simulink model "hk_ac_elec_load_rt_2024b"  (R2024b)
settings: Solver=FixedStepAuto  StartTime=0.0  StopTime=inf  FixedStep=1  RelTol=1e-3
libraries: Links_CHRU34207S_Lib x32, simulink x1
settings Model: Creator=Administrator  LastModifiedBy=gao
settings OptimizationCC: BlockReduction=off  ReuseModelBlockBuffer=off
settings HardwareCC: ProdBitPerLong=64  ProdHWDeviceType=Intel->x86-64 (Linux 64)
settings RTWCC: SystemTargetFile=links_rtlnx_grt.tlc  TemplateMakefile=links_rtlnx_grt.tmf  GPUComputeCapability=3.5
settings STFCustomTargetCC: TargetLangStandard=C99 (ISO)  CombineOutputUpdateFcns=on  SystemTargetFile=links_rtlnx_grt.tlc
settings GRTTargetCC: ParMdlRefBuildCompliant=off  CompOptLevelCompliant=off  ConcurrentExecutionCompliant=off  MatFileLogging=off  CPPClassGenCompliant=off  UseToolchainInfoCompliant=off  RTWCAPISignals=on  RTWCAPIParams=on  RTWCAPIRootIO=on
settings ConfigComp: CovMetricSettings=de  CovBoundaryAbsTol=1.0e-5

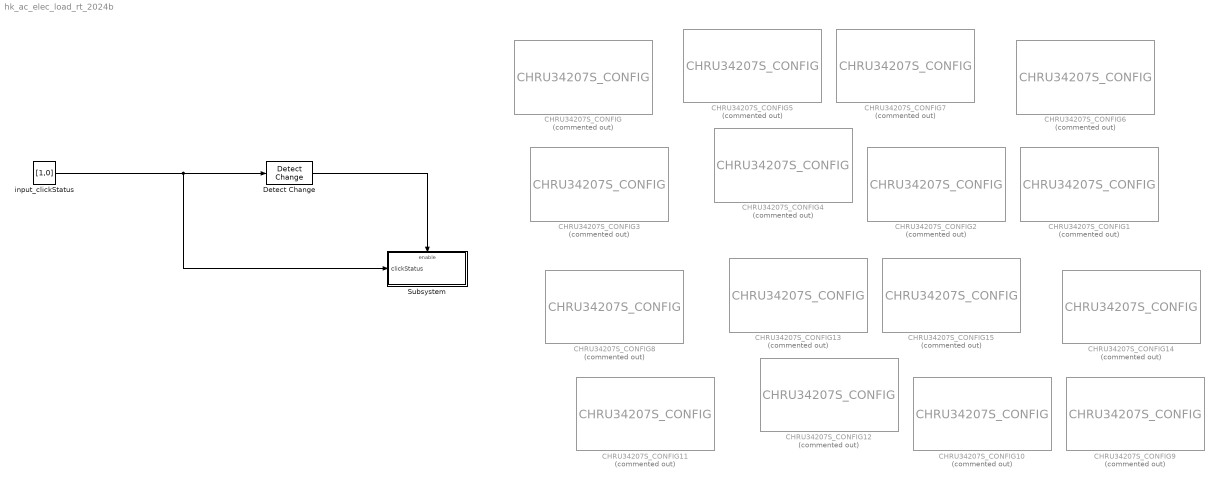
== system hk_ac_elec_load_rt_2024b ==
  CHRU34207S_CONFIG : Links_CHRU34207S_Lib/CHRU34207S_CONFIG  Commented=on  Card=0  Channel=0  Mode=RS422  Baud=115200  Parity=None  DataBits=8  StopBits=1  SampleTime=-1
      settings: SourceProductName=Links_LnxLib
  CHRU34207S_CONFIG1 : Links_CHRU34207S_Lib/CHRU34207S_CONFIG  Commented=on  Card=0  Channel=7  Mode=RS422  Baud=115200  Parity=None  DataBits=8  StopBits=1  SampleTime=-1
      settings: SourceProductName=Links_LnxLib
  CHRU34207S_CONFIG10 : Links_CHRU34207S_Lib/CHRU34207S_CONFIG  Commented=on  Card=0  Channel=14  Mode=RS422  Baud=115200  Parity=None  DataBits=8  StopBits=1  SampleTime=-1
      settings: SourceProductName=Links_LnxLib
  CHRU34207S_CONFIG11 : Links_CHRU34207S_Lib/CHRU34207S_CONFIG  Commented=on  Card=0  Channel=12  Mode=RS422  Baud=115200  Parity=None  DataBits=8  StopBits=1  SampleTime=-1
      settings: SourceProductName=Links_LnxLib
  CHRU34207S_CONFIG12 : Links_CHRU34207S_Lib/CHRU34207S_CONFIG  Commented=on  Card=0  Channel=13  Mode=RS422  Baud=115200  Parity=None  DataBits=8  StopBits=1  SampleTime=-1
      settings: SourceProductName=Links_LnxLib
  CHRU34207S_CONFIG13 : Links_CHRU34207S_Lib/CHRU34207S_CONFIG  Commented=on  Card=0  Channel=9  Mode=RS422  Baud=115200  Parity=None  DataBits=8  StopBits=1  SampleTime=-1
      settings: SourceProductName=Links_LnxLib
  CHRU34207S_CONFIG14 : Links_CHRU34207S_Lib/CHRU34207S_CONFIG  Commented=on  Card=0  Channel=11  Mode=RS422  Baud=115200  Parity=None  DataBits=8  StopBits=1  SampleTime=-1
      settings: SourceProductName=Links_LnxLib
  CHRU34207S_CONFIG15 : Links_CHRU34207S_Lib/CHRU34207S_CONFIG  Commented=on  Card=0  Channel=10  Mode=RS422  Baud=115200  Parity=None  DataBits=8  StopBits=1  SampleTime=-1
      settings: SourceProductName=Links_LnxLib
  CHRU34207S_CONFIG2 : Links_CHRU34207S_Lib/CHRU34207S_CONFIG  Commented=on  Card=0  Channel=6  Mode=RS422  Baud=115200  Parity=None  DataBits=8  StopBits=1  SampleTime=-1
      settings: SourceProductName=Links_LnxLib
  CHRU34207S_CONFIG3 : Links_CHRU34207S_Lib/CHRU34207S_CONFIG  Commented=on  Card=0  Channel=4  Mode=RS422  Baud=115200  Parity=None  DataBits=8  StopBits=1  SampleTime=-1
      settings: SourceProductName=Links_LnxLib
  CHRU34207S_CONFIG4 : Links_CHRU34207S_Lib/CHRU34207S_CONFIG  Commented=on  Card=0  Channel=5  Mode=RS422  Baud=115200  Parity=None  DataBits=8  StopBits=1  SampleTime=-1
      settings: SourceProductName=Links_LnxLib
  CHRU34207S_CONFIG5 : Links_CHRU34207S_Lib/CHRU34207S_CONFIG  Commented=on  Card=0  Channel=1  Mode=RS422  Baud=115200  Parity=None  DataBits=8  StopBits=1  SampleTime=-1
      settings: SourceProductName=Links_LnxLib
  CHRU34207S_CONFIG6 : Links_CHRU34207S_Lib/CHRU34207S_CONFIG  Commented=on  Card=0  Channel=3  Mode=RS422  Baud=115200  Parity=None  DataBits=8  StopBits=1  SampleTime=-1
      settings: SourceProductName=Links_LnxLib
  CHRU34207S_CONFIG7 : Links_CHRU34207S_Lib/CHRU34207S_CONFIG  Commented=on  Card=0  Channel=2  Mode=RS422  Baud=115200  Parity=None  DataBits=8  StopBits=1  SampleTime=-1
      settings: SourceProductName=Links_LnxLib
  CHRU34207S_CONFIG8 : Links_CHRU34207S_Lib/CHRU34207S_CONFIG  Commented=on  Card=0  Channel=8  Mode=RS422  Baud=115200  Parity=None  DataBits=8  StopBits=1  SampleTime=-1
      settings: SourceProductName=Links_LnxLib
  CHRU34207S_CONFIG9 : Links_CHRU34207S_Lib/CHRU34207S_CONFIG  Commented=on  Card=0  Channel=15  Mode=RS422  Baud=115200  Parity=None  DataBits=8  StopBits=1  SampleTime=-1
      settings: SourceProductName=Links_LnxLib
  Detect Change : simulink/Logic and Bit Operations/Detect Change  vinit=[0,0]  OutDataTypeStr=boolean
  Subsystem : Subsystem
  input_clickStatus : Constant  Value=[1,0]  VectorParams1D=off
  wires:
  input_clickStatus/1 -> Subsystem/1(clickStatus), Detect Change/1
  Detect Change/1 -> Subsystem/Enable

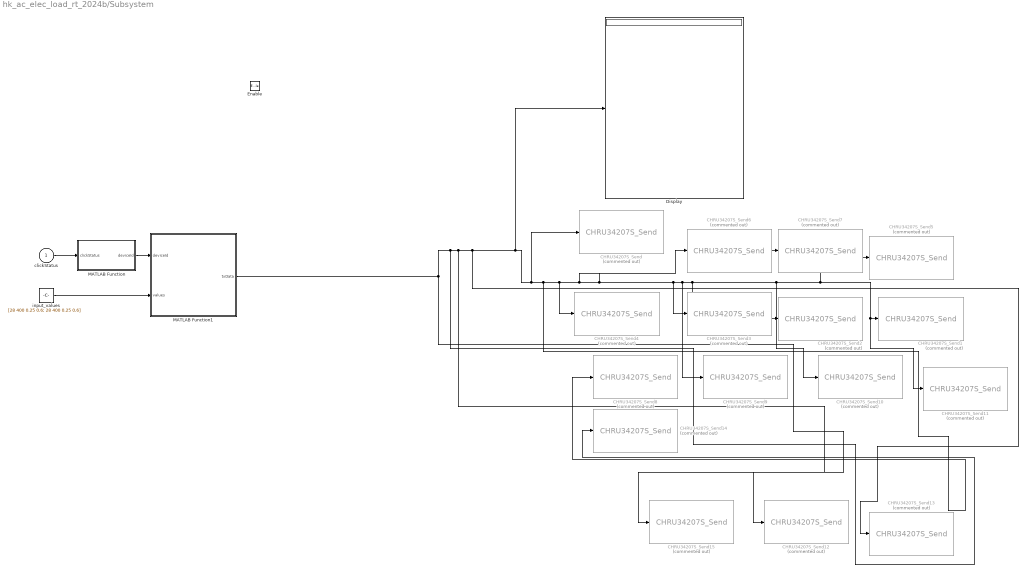
== system hk_ac_elec_load_rt_2024b/Subsystem ==
  clickStatus : Inport
  Enable : EnablePort
  CHRU34207S_Send : Links_CHRU34207S_Lib/CHRU34207S_Send  Commented=on  Card=0  Channel=0  SampleTime=-1
      settings: SourceProductName=Links_LnxLib
  CHRU34207S_Send1 : Links_CHRU34207S_Lib/CHRU34207S_Send  Commented=on  Card=0  Channel=7  SampleTime=-1
      settings: SourceProductName=Links_LnxLib
  CHRU34207S_Send10 : Links_CHRU34207S_Lib/CHRU34207S_Send  Commented=on  Card=0  Channel=10  SampleTime=-1
      settings: SourceProductName=Links_LnxLib
  CHRU34207S_Send11 : Links_CHRU34207S_Lib/CHRU34207S_Send  Commented=on  Card=0  Channel=11  SampleTime=-1
      settings: SourceProductName=Links_LnxLib
  CHRU34207S_Send12 : Links_CHRU34207S_Lib/CHRU34207S_Send  Commented=on  Card=0  Channel=14  SampleTime=-1
      settings: SourceProductName=Links_LnxLib
  CHRU34207S_Send13 : Links_CHRU34207S_Lib/CHRU34207S_Send  Commented=on  Card=0  Channel=15  SampleTime=-1
      settings: SourceProductName=Links_LnxLib
  CHRU34207S_Send14 : Links_CHRU34207S_Lib/CHRU34207S_Send  Commented=on  Card=0  Channel=12  SampleTime=-1
      settings: SourceProductName=Links_LnxLib
  CHRU34207S_Send15 : Links_CHRU34207S_Lib/CHRU34207S_Send  Commented=on  Card=0  Channel=13  SampleTime=-1
      settings: SourceProductName=Links_LnxLib
  CHRU34207S_Send2 : Links_CHRU34207S_Lib/CHRU34207S_Send  Commented=on  Card=0  Channel=6  SampleTime=-1
      settings: SourceProductName=Links_LnxLib
  CHRU34207S_Send3 : Links_CHRU34207S_Lib/CHRU34207S_Send  Commented=on  Card=0  Channel=5  SampleTime=-1
      settings: SourceProductName=Links_LnxLib
  CHRU34207S_Send4 : Links_CHRU34207S_Lib/CHRU34207S_Send  Commented=on  Card=0  Channel=4  SampleTime=-1
      settings: SourceProductName=Links_LnxLib
  CHRU34207S_Send5 : Links_CHRU34207S_Lib/CHRU34207S_Send  Commented=on  Card=0  Channel=3  SampleTime=-1
      settings: SourceProductName=Links_LnxLib
  CHRU34207S_Send6 : Links_CHRU34207S_Lib/CHRU34207S_Send  Commented=on  Card=0  Channel=1  SampleTime=-1
      settings: SourceProductName=Links_LnxLib
  CHRU34207S_Send7 : Links_CHRU34207S_Lib/CHRU34207S_Send  Commented=on  Card=0  Channel=2  SampleTime=-1
      settings: SourceProductName=Links_LnxLib
  CHRU34207S_Send8 : Links_CHRU34207S_Lib/CHRU34207S_Send  Commented=on  Card=0  Channel=8  SampleTime=-1
      settings: SourceProductName=Links_LnxLib
  CHRU34207S_Send9 : Links_CHRU34207S_Lib/CHRU34207S_Send  Commented=on  Card=0  Channel=9  SampleTime=-1
      settings: SourceProductName=Links_LnxLib
  Display : Display
      settings: Format=hex (Stored Integer)
  MATLAB Function : MATLAB Function  TreatAsAtomicUnit=on
  MATLAB Function1 : MATLAB Function  TreatAsAtomicUnit=on
  input_values : Constant  Value=[28 400 0.25 0.6; 28 400 0.25 0.6]  VectorParams1D=off
  wires:
  input_values/1 -> MATLAB Function1/2(values)
  MATLAB Function1/1(txData) -> CHRU34207S_Send15/1, CHRU34207S_Send13/1, CHRU34207S_Send/1, CHRU34207S_Send8/1, CHRU34207S_Send4/1, CHRU34207S_Send6/1, CHRU34207S_Send7/1, CHRU34207S_Send9/1, CHRU34207S_Send2/1, CHRU34207S_Send10/1, CHRU34207S_Send11/1, CHRU34207S_Send1/1, CHRU34207S_Send5/1, CHRU34207S_Send3/1, Display/1, CHRU34207S_Send14/1, CHRU34207S_Send12/1
  clickStatus/1 -> MATLAB Function/1(clickStatus)
  MATLAB Function/1(deviceId) -> MATLAB Function1/1(deviceId)

== matlab function hk_ac_elec_load_rt_2024b/Subsystem/MATLAB Function1 ==
  data: deviceId input; values input; txData output
function txData  = ac_load_cmd_gene(deviceId,values)
% values: 2行4列
% 每行: [V, f, I, PF]
% ✅ 统一初始化输出
FRAME_LEN = 22;
txData = zeros(1, FRAME_LEN, 'uint8');

% 参数对象
p = acload_params();

% 设备数量由 values 行数决定（代码生成时可固定为 2）
numDevices = 2;

for k = 1:numDevices
    p.devices(k).V_rms      = values(k,1);
    p.devices(k).f_Hz       = values(k,2);
    p.devices(k).I_target_A = values(k,3);
    p.devices(k).PF_target  = values(k,4);
end

% 求解全部设备
results = acload_relay([], p);

frame = acload_frame(results.devices(deviceId).data);
txData(1:FRAME_LEN) = frame(1:FRAME_LEN);

end

function params = acload_params()
%ACLOAD_PARAMS 两台交流电子负载的实测参数配置
%
% 单位：
%   V_rms、I_target_A：V、A
%   f_Hz：Hz
%   R0_ohm、R_ohm、Rser_ohm、Lser_ohm：ohm
%   Ls_H、L_H：H
%
% 实测工况（数字电桥；对应表内行标题）：
%   R0        ：固定电阻单独测量。
%   R1~R10    ：电感全接（11 节全部串入）、只接一只电阻 → 读数 = R0∥Ri + 电感链内阻。
%   Rs        ：电阻全接、电感全接 → 读数 = R0∥R1∥…∥R10 + 电感链内阻。
%   Ls        ：电阻全接、电感全断（全部被短接）→ 仅剩线路寄生电感。
%   L1~L11    ：电阻全接、只接一只电感 → 读数 = Lj + Ls。
%
% 反推（记 d = 11 节电感全部投入时的总线内阻）：
%   由单只电阻读数：1/Ri = 1/(Ri_meas-d) - 1/R0
%   代入 Rs：Rs = d + 1/( Σ 1/(Ri_meas-d) - 9/R0 )
%   其中 Σ 为 i=1,...,10。
%   注意：每项 1/(Ri_meas-d) 已经包含一份 1/R0；10 项求和后包含 10/R0，
%         实际电路中固定电阻 R0 只出现一次，因此应减去 9/R0。
%         不能再额外加 1/R0，否则会重复计入 R0。
%   电感：Lj = Lj_meas - Ls（Ls 只减一次，且始终在回路里，求解时再加回一次）。
%   电阻：Ri = 1/( 1/(Ri_meas-d) - 1/R0 )。
%   校验：Rser 由未四舍五入的原始测量值反求；文件中的 R_ohm 保留两位小数，
%         因此直接用本文件数组回算 Rs 会有舍入误差（六组最大约 0.0006 ohm）。
%         六组实测 Rs 分别为：5.070 / 4.833 / 4.780 / 6.600 / 6.600 / 6.600 ohm。
%
% Lser_ohm（逐节电感自身的内阻，1×11）：
%   电感继电器闭合会把该节线圈连同其铜阻一起旁路，所以回路里真正存在的串联内阻
%   是 Σ(投入那几节的内阻)，不是整条链的 d。逐节值按 r_j ∝ L_j 由 d 分摊，和为 d，
%   因此"全接"时复现 Rs、"全断"时只剩线路/触点等未建模电阻（此处忽略）。
%   这仍是对 r_j 的假设；若日后用万用表测得每节电感的直流电阻，直接替换该数组即可，
%   求解程序无需改动。删掉 Lser_ohm 则退化为"整链 d 恒定串联"的近似。
%
% 继电器语义：
%   电阻继电器 CLOSED：对应电阻投入并联网络。
%   电感继电器 CLOSED：对应电感被短接；OPEN：对应电感计入串联链。

%% 预分配设备结构体数组（避免 Simulink 索引报错）
device1 = struct();
device2 = struct();

%% ===== 设备1 =====
device1.id = 1;
device1.name = 'device1';
device1.V_rms = 28;
device1.f_Hz = 400;
device1.I_target_A = 0.25;
device1.PF_target = 0.6;

% 第1组
g1 = struct();
g1.id = 1;
g1.R0_ohm = 1005.0;
g1.Rser_ohm = 0.6519527417;
g1.Ls_H = 6.7e-6;
g1.R_ohm = [407.12, 204.68, 102.91, 102.91, 102.78, 102.66, 22.33, 22.33, 22.33, 22.33];
g1.L_H = [0.10460, 0.19830, 0.39830, 0.80380, 1.62330, 3.04330, 5.67830, 9.92030, 10.09330, 10.11330, 19.97130] * 1e-3;
g1.Lser_ohm = [0.00110083, 0.00208694, 0.00419178, 0.00845933, 0.0170839, 0.0320282, 0.0597594, 0.104403, 0.106224, 0.106434, 0.210181];

% 第2组
g2 = struct();
g2.id = 2;
g2.R0_ohm = 998.5;
g2.Rser_ohm = 0.3620498265;
g2.Ls_H = 6.93e-6;
g2.R_ohm = [405.61, 204.21, 102.84, 103.08, 102.84, 103.33, 22.64, 22.64, 22.64, 22.74];
g2.L_H = [0.10457, 0.20847, 0.40107, 0.77577, 1.57207, 2.97107, 5.57807, 9.95307, 9.91307, 10.09307, 20.03307] * 1e-3;
g2.Lser_ohm = [0.000614569, 0.0012252, 0.00235713, 0.00455929, 0.00923923, 0.0174613, 0.0327829, 0.0584953, 0.0582602, 0.0593181, 0.117737];

% 第3组
g3 = struct();
g3.id = 3;
g3.R0_ohm = 992.2;
g3.Rser_ohm = 0.2972979542;
g3.Ls_H = 6.88e-6;
g3.R_ohm = [405.19, 204.72, 103.47, 102.99, 103.23, 103.35, 22.66, 23.06, 22.79, 22.42];
g3.L_H = [0.09242, 0.18872, 0.39052, 0.79372, 1.55562, 2.98012, 5.58812, 9.95812, 9.96812, 9.89612, 20.01312] * 1e-3;
g3.Lser_ohm = [0.000447316, 0.000913412, 0.00189013, 0.00384163, 0.00752926, 0.0144239, 0.0270467, 0.0481977, 0.0482461, 0.0478976, 0.0968643];

device1.groups = [g1, g2, g3];

%% ===== 设备2 =====
device2.id = 2;
device2.name = 'device2';
device2.V_rms = 28;
device2.f_Hz = 400;
device2.I_target_A = 0.25;
device2.PF_target = 0.6;

% 第1组
g1 = struct();
g1.id = 1;
g1.R0_ohm = 998.3;
g1.Rser_ohm = 2.559091505;
g1.Ls_H = 6.7e-6;
g1.R_ohm = [399.15, 200.90, 100.42, 100.30, 100.42, 100.42, 20.04, 20.14, 20.24, 19.93];
g1.L_H = [0.09400, 0.18890, 0.38270, 0.78230, 1.56170, 2.95100, 5.97330, 10.00930, 9.94030, 10.01130, 19.99330] * 1e-3;
g1.Lser_ohm = [0.00388693, 0.00781107, 0.0158248, 0.0323483, 0.0645768, 0.122025, 0.246998, 0.413888, 0.411034, 0.41397, 0.826729];

% 第2组
g2 = struct();
g2.id = 2;
g2.R0_ohm = 995.5;
g2.Rser_ohm = 2.571286619;
g2.Ls_H = 6.65e-6;
g2.R_ohm = [399.18, 200.27, 100.31, 99.95, 100.07, 100.19, 20.02, 19.97, 19.97, 20.13];
g2.L_H = [0.09495, 0.19185, 0.38735, 0.77855, 1.59335, 2.98935, 5.57035, 9.97635, 9.92135, 9.88335, 19.73935] * 1e-3;
g2.Lser_ohm = [0.0039941, 0.00807022, 0.016294, 0.0327499, 0.0670247, 0.125748, 0.234318, 0.419658, 0.417344, 0.415746, 0.830341];

% 第3组
g3 = struct();
g3.id = 3;
g3.R0_ohm = 995.7;
g3.Rser_ohm = 2.550334502;
g3.Ls_H = 6.9e-6;
g3.R_ohm = [399.19, 200.44, 99.73, 100.46, 100.33, 100.33, 20.15, 20.25, 20.15, 20.05];
g3.L_H = [0.09770, 0.19430, 0.38310, 0.78340, 1.57910, 2.96310, 5.52010, 10.03510, 9.77310, 10.02910, 20.01310] * 1e-3;
g3.Lser_ohm = [0.00406001, 0.00807431, 0.0159201, 0.0325549, 0.0656209, 0.123134, 0.229393, 0.417017, 0.40613, 0.416768, 0.831662];

device2.groups = [g1, g2, g3];

%% 最终输出
params = struct();
params.devices = [device1, device2];

end
function results = acload_relay(deviceId, params)
%ACLOAD_RELAY 求解两台交流电子负载各组的最优继电器开合状态
%
% 用法：
%   results = acload_relay();          % 读取 acload_params.m，求解全部设备
%   results = acload_relay(1);         % 只求解设备 ID=1
%   results = acload_relay(2);         % 只求解设备 ID=2
%   p = acload_params();
%   results = acload_relay([], p);     % 使用自定义参数，求解全部设备
%   results = acload_relay(2, p);      % 使用自定义参数，只求解设备 ID=2
%   注：代码生成下不支持 acload_relay(p) 这种单 struct 入参重载，
%       自定义参数一律写成双入参 acload_relay([], p)。
%
% 参数结构与 acload_params.m 一致：
%   params.devices(k).V_rms / f_Hz / I_target_A / PF_target
%   params.devices(k).groups(g).R0_ohm / R_ohm / Ls_H / L_H
%   可选字段：Rser_ohm、Lser_ohm
%
% 电路模型：
%   1) R0 固定接入；R1~R10 通过继电器并联投入。
%   2) L1~L11 串联；电感继电器 CLOSED 时，该节电感及其绕组电阻均被旁路。
%   3) Ls_H 是线路寄生电感，始终计入总电感，即使所有电感均被旁路。
%   4) 若存在 Lser_ohm，按实际投入的电感节累加绕组电阻；不再额外叠加
%      Rser_ohm，避免重复计算。Lser_ohm 的逐节分配目前是参数文件中的估算值。
%      若没有 Lser_ohm、但有 Rser_ohm，则将 Rser_ohm 作为恒定串联电阻近似。
%
% 优化目标（电流和功率因数权重0.8和0.2）：
%   J = 0.8*((I-I_target)/I_target)^2 + 0.2*((PF-PF_target)/PF_target)^2
%
% 每组完整穷举 2^10 种电阻状态 × 2^11 种电感状态，共 2,097,152 种组合。
%
% 继电器状态语义：
%   resistorRelayClosed(j) = true  -> Rj 继电器闭合，电阻投入并联网络。
%   inductorRelayClosed(j) = true  -> Lj 继电器闭合，电感及其绕组电阻被短接。
%
% 控制数据输出：
%   results.devices(k).data 为第 k 台设备的16字节控制数据。
%   通信组1~3对应优化组1~3，通信组4的继电器控制位填0。
%   每组4字节，按小端序排列。
%
% 通信组32位定义（位编号从Bit0开始）：
%   Bit0~1   ：组号，组1~4依次为00、01、10、11
%   Bit2~11 ：R1~R10
%   Bit12~13：预留，填0
%   Bit14~24：L1~L11
%   Bit25~31：预留，填0

%% 解析输入参数
% 代码生成约束：deviceId 始终是数值标量或空 double，params 始终是结构体，
% 不再提供"单个 struct 入参"重载，以免同一变量在分支里被改类型。
if nargin < 1
    deviceId = [];
end
if nargin < 2
    params = acload_params();
end

validate_device_collection(params);
allIds = [params.devices.id];

if isempty(deviceId)
    selectedIndices = 1:numel(params.devices);
else
    if ~isnumeric(deviceId) || ~isreal(deviceId) || ...
            ~isscalar(deviceId) || isnan(deviceId) || ...
            isinf(deviceId) || deviceId ~= fix(deviceId)
        error('acload_relay:InvalidDeviceId', ...
            'deviceId must be an integer device ID, or empty to solve all devices.');
    end
    selectedIndices = 0;
    for k = 1:numel(allIds)
        if allIds(k) == deviceId
            selectedIndices = k;
        end
    end
    if selectedIndices == 0
        error('acload_relay:UnknownDeviceId', ...
            'Device ID %g does not exist in the parameters.', deviceId);
    end
end

%% 预生成所有继电器状态组合
nR = 10;
nL = 11;
nRComb = 2^nR;
nLComb = 2^nL;

% 电阻位为 true 表示继电器闭合、该电阻投入。
rMask = uint16((0:nRComb-1)');
rClosedBits = false(nRComb, nR);
for k = 1:nR
    rClosedBits(:, k) = bitget(rMask, k) ~= 0;
end

% 电感位为 true 表示电感计入串联链（即对应继电器断开）。
lMask = uint16((0:nLComb-1)');
lIncludedBits = false(nLComb, nL);
for k = 1:nL
    lIncludedBits(:, k) = bitget(lMask, k) ~= 0;
end

%% 结果结构体模板
% 代码生成约束：结构体字段不得含 cell / 变长 char，只保留定长数值与逻辑字段。
emptyGroup = struct( ...
    'resistorRelayClosed', false(1, nR), ...
    'inductorRelayClosed', false(1, nL), ...
    'parallelResistanceOhm', NaN, ...
    'inductorWindingResistanceOhm', NaN, ...
    'equivalentResistanceOhm', NaN, ...
    'totalInductanceH', NaN, ...
    'inductiveReactanceOhm', NaN, ...
    'impedanceMagnitudeOhm', NaN, ...
    'currentRmsA', NaN, ...
    'powerFactor', NaN, ...
    'realPowerW', NaN, ...
    'objectiveJ', NaN);

% 代码生成约束：去掉变长 char 字段与嵌套 struct 数组字段（仅用于回看，不参与输出）。
emptyDevice = struct( ...
    'deviceId', NaN, ...
    'V_rms', NaN, ...
    'f_Hz', NaN, ...
    'I_target_A', NaN, ...
    'PF_target', NaN, ...
    'data', zeros(1, 16, 'uint8'));

% 代码生成约束：结构体必须一次性定义全部字段，且数组长度固定。
% 主函数只读取 results.devices(2).data；无参调用时两台设备都会被求解，
% 故 devices 固定为 1x2，与原 acload_relay() 行为一致。
results = struct( ...
    'devices', repmat(emptyDevice, 1, 2));

%% 逐台设备、逐组求最优继电器状态
for outputIndex = 1:numel(selectedIndices)
    deviceIndex = selectedIndices(outputIndex);
    device = params.devices(deviceIndex);
    validate_one_device(device, deviceIndex);

    omega = 2 * pi * device.f_Hz;
    groupResults = repmat(emptyGroup, 1, 3);

    %% 逐组优化
    for groupIndex = 1:3
        g = device.groups(groupIndex);
        R_values = g.R_ohm(:);
        L_values = g.L_H(:);

        %% A. 计算所有电阻继电器组合的并联等效电阻
        % R_parallel = 1 / (1/R0 + sum(closed_Rj / Rj))
        conductanceAll = 1 / g.R0_ohm + ...
            double(rClosedBits) * (1 ./ R_values);
        R_parallel_all = 1 ./ conductanceAll;

        %% B. 计算所有电感组合的总电感和绕组串联电阻
        % lIncludedBits=true 表示该节线圈投入；
        % 其电感及铜阻均计入。
        L_active_all = double(lIncludedBits) * L_values;
        L_total_all = g.Ls_H + L_active_all;

        if isfield(g, 'Lser_ohm') && ~isempty(g.Lser_ohm)
            % 逐节模型：继电器短接哪一节，该节绕组电阻也同时旁路。
            R_winding_all = double(lIncludedBits) * g.Lser_ohm(:);
%             windingModel = 'per-section Lser_ohm';  % 仅用于已注释的打印
        elseif isfield(g, 'Rser_ohm') && ~isempty(g.Rser_ohm)
            % 退化近似：没有逐节电阻数据时，
            % 将整链内阻视为恒定串联电阻。
            R_winding_all = repmat(g.Rser_ohm, nLComb, 1);
%             windingModel = 'constant Rser_ohm approximation';  % 仅用于已注释的打印
        else
            R_winding_all = zeros(nLComb, 1);
%             windingModel = 'inductor winding resistance not included';  % 仅用于已注释的打印
        end

        X_L_all = omega .* L_total_all;

        %% C. 穷举全部电阻×电感组合
        bestJ = inf;
        bestRIndex = 1;
        bestLIndex = 1;
        bestCurrent = NaN;
        bestPF = NaN;
        bestRTotal = NaN;
        bestZ = NaN;

        for rIndex = 1:nRComb
            % 总串联电阻 = 电阻并联网络等效电阻
            % + 当前投入电感的绕组电阻。
            R_total_all = R_parallel_all(rIndex) + R_winding_all;
            Z_abs_all = sqrt(R_total_all.^2 + X_L_all.^2);
            currentAll = device.V_rms ./ Z_abs_all;
            PF_all = R_total_all ./ Z_abs_all;

            % 电流误差权重80%，功率因数误差权重20%。
            J_all = ...
                0.8 * ((currentAll - device.I_target_A) ./ ...
                device.I_target_A).^2 + ...
                0.2 * ((PF_all - device.PF_target) ./ ...
                device.PF_target).^2;

            [localBestJ, lIndex] = min(J_all);
            if localBestJ < bestJ
                bestJ = localBestJ;
                bestRIndex = rIndex;
                bestLIndex = lIndex;
                bestCurrent = currentAll(lIndex);
                bestPF = PF_all(lIndex);
                bestRTotal = R_total_all(lIndex);
                bestZ = Z_abs_all(lIndex);
            end
        end

        %% D. 保存该组最优状态和预测结果
        resistorClosed = rClosedBits(bestRIndex, :);
        % CLOSED=短接，因此取反得到继电器闭合状态。
        inductorClosed = ~lIncludedBits(bestLIndex, :);

        bestRparallel = R_parallel_all(bestRIndex);
        bestRwinding = R_winding_all(bestLIndex);
        bestLtotal = L_total_all(bestLIndex);
        bestX = omega * bestLtotal;
        bestP = bestCurrent^2 * bestRTotal;

        oneGroup = emptyGroup;
        oneGroup.resistorRelayClosed = resistorClosed;
        oneGroup.inductorRelayClosed = inductorClosed;
        oneGroup.parallelResistanceOhm = bestRparallel;
        oneGroup.inductorWindingResistanceOhm = bestRwinding;
        oneGroup.equivalentResistanceOhm = bestRTotal;
        oneGroup.totalInductanceH = bestLtotal;
        oneGroup.inductiveReactanceOhm = bestX;
        oneGroup.impedanceMagnitudeOhm = bestZ;
        oneGroup.currentRmsA = bestCurrent;
        oneGroup.powerFactor = bestPF;
        oneGroup.realPowerW = bestP;
        oneGroup.objectiveJ = bestJ;
        groupResults(groupIndex) = oneGroup;

        %% 输出计算结果
%         fprintf('\n--- %s 第%d组计算完成（%s）---\n', ...
%             get_device_name(device, deviceIndex), groupIndex, windingModel);
%         fprintf('  预测电流 I       = %.9g A rms（目标 %.9g A）\n', ...
%             bestCurrent, device.I_target_A);
%         fprintf('  预测功率因数 PF  = %.9g（目标 %.9g）\n', ...
%             bestPF, device.PF_target);
%         fprintf('  并联电阻 Rparallel = %.9g ohm\n', bestRparallel);
%         fprintf('  电感绕组电阻      = %.9g ohm\n', bestRwinding);
%         fprintf('  总等效电阻 Rtotal = %.9g ohm\n', bestRTotal);
%         fprintf('  总电感 Ltotal     = %.9g mH（含 Ls）\n', ...
%             bestLtotal * 1e3);
%         fprintf('  感抗 X_L           = %.9g ohm\n', bestX);
%         fprintf('  阻抗幅值 |Z|       = %.9g ohm\n', bestZ);
%         fprintf('  有功功率 P         = %.9g W\n', bestP);
%         fprintf('  目标函数 J         = %.12g\n', bestJ);
%         fprintf('  电阻继电器 R1~R10（CLOSED=投入）：%s\n', ...
%             sprintf('%d ', resistorClosed));
%         fprintf('  电感继电器 L1~L11（CLOSED=短接）：%s\n', ...
%             sprintf('%d ', inductorClosed));
    end

    %% E. 将本设备3组继电器状态转换为16字节控制数据
    % 通信组1~3映射优化组1~3。
    % 通信组4为预留组，继电器控制位全部填0。
    deviceData = zeros(1, 16, 'uint8');

    for controlGroupIndex = 1:4
        if controlGroupIndex <= 3
            rClosed = groupResults(controlGroupIndex).resistorRelayClosed;
            lClosed = groupResults(controlGroupIndex).inductorRelayClosed;
        else
            % 通信组4没有对应的优化组，继电器控制位填0。
            rClosed = false(1, 10);
            lClosed = false(1, 11);
        end

        % 32位组字。
        % Bit0~1：组号。
        % Bit2~11：R1~R10。
        % Bit12~13：预留。
        % Bit14~24：L1~L11。
        % Bit25~31：预留。
        groupWord = uint32(controlGroupIndex - 1);

        %% 写入电阻继电器状态
        for relayIndex = 1:10
            if rClosed(relayIndex)
                % R1对应Bit2，R2对应Bit3，依此类推。
                groupWord = bitset(groupWord, 2 + relayIndex, 1);
            end
        end

        %% 写入电感继电器状态
        for relayIndex = 1:11
            if lClosed(relayIndex)
                % L1对应Bit14，L2对应Bit15，依此类推。
                groupWord = bitset(groupWord, 14 + relayIndex, 1);
            end
        end

        %% 按小端序拆分为4字节
        % 低字节在前，高字节在后。
        byteOffset = (controlGroupIndex - 1) * 4;
        for byteIndex = 0:3
            deviceData(byteOffset + byteIndex + 1) = ...
                uint8(bitand( ...
                bitshift(groupWord, -8 * byteIndex), ...
                uint32(255)));
        end
    end

    %% F. 保存设备计算结果和控制数据
    oneDevice = emptyDevice;
    oneDevice.deviceId = device.id;
%     oneDevice.name = get_device_name(device, deviceIndex);  % 展示字段，代码生成不适用
    oneDevice.V_rms = device.V_rms;
    oneDevice.f_Hz = device.f_Hz;
    oneDevice.I_target_A = device.I_target_A;
    oneDevice.PF_target = device.PF_target;
%     oneDevice.groups = groupResults;  % 嵌套 struct 数组，仅用于回看
    % 每台设备自己的16字节控制数据。
    oneDevice.data = deviceData;
    results.devices(outputIndex) = oneDevice;

    %% 输出控制数据
%     fprintf('\n--- %s 控制数据（16字节，小端序）---\n', oneDevice.name);
%     fprintf('  ');
%     fprintf('%02X ', deviceData);
%     fprintf('\n');
end
end

function validate_device_collection(p)
% 检查设备集合结构，以及设备编号是否唯一。
if ~isstruct(p) || ~isfield(p, 'devices') || ...
        ~isstruct(p.devices) || isempty(p.devices)
    error('acload_relay:InvalidParameters', ...
        'params must contain a non-empty struct array params.devices.');
end
if ~isfield(p.devices, 'id')
    error('acload_relay:MissingDeviceId', ...
        'Each device must define an id.');
end
ids = zeros(1, numel(p.devices));
for k = 1:numel(p.devices)
    id = p.devices(k).id;
    if ~is_positive_integer_scalar(id)
        error('acload_relay:InvalidDeviceId', ...
            'The id of device %d must be a positive integer.', k);
    end
    ids(k) = id;
end
for a = 1:numel(ids)
    for b = a+1:numel(ids)
        if ids(a) == ids(b)
            error('acload_relay:DuplicateDeviceId', ...
                'IDs in params.devices must be unique.');
        end
    end
end
end

function validate_one_device(d, deviceIndex)
% 检查单台设备的电源目标和三组器件参数。
if ~isfield(d, 'V_rms') || ~is_positive_finite_scalar(d.V_rms)
    error('acload_relay:InvalidVoltage', ...
        'V_rms of device %d must be a finite positive scalar.', deviceIndex);
end
if ~isfield(d, 'f_Hz') || ~is_positive_finite_scalar(d.f_Hz)
    error('acload_relay:InvalidFrequency', ...
        'f_Hz of device %d must be a finite positive scalar.', deviceIndex);
end
if ~isfield(d, 'I_target_A') || ...
        ~is_positive_finite_scalar(d.I_target_A)
    error('acload_relay:InvalidTargetCurrent', ...
        'I_target_A of device %d must be a finite positive scalar.', deviceIndex);
end
if ~isfield(d, 'PF_target') || ...
        ~is_positive_finite_scalar(d.PF_target) || ...
        d.PF_target > 1
    error('acload_relay:InvalidTargetPF', ...
        'PF_target of device %d must satisfy 0 < PF_target <= 1.', deviceIndex);
end
if ~isfield(d, 'groups') || ...
        ~isstruct(d.groups) || numel(d.groups) ~= 3
    error('acload_relay:InvalidGroups', ...
        'groups of device %d must contain exactly 3 groups.', deviceIndex);
end
for groupIndex = 1:3
    g = d.groups(groupIndex);
    if ~isfield(g, 'R0_ohm') || ...
            ~is_positive_finite_scalar(g.R0_ohm)
        error('acload_relay:InvalidR0', ...
            'R0_ohm of device %d group %d must be a finite positive scalar.', ...
            deviceIndex, groupIndex);
    end
    if ~isfield(g, 'R_ohm') || ...
            ~is_positive_finite_vector(g.R_ohm, 10)
        error('acload_relay:InvalidResistors', ...
            'R_ohm of device %d group %d must contain 10 finite positive values.', ...
            deviceIndex, groupIndex);
    end
    if ~isfield(g, 'L_H') || ...
            ~is_positive_finite_vector(g.L_H, 11)
        error('acload_relay:InvalidInductors', ...
            ['L_H of device %d group %d must contain 11 finite positive values' ...
            ' (unit H).'], deviceIndex, groupIndex);
    end
    if ~isfield(g, 'Ls_H') || ...
            ~is_nonnegative_finite_scalar(g.Ls_H)
        error('acload_relay:InvalidLineInductance', ...
            'Ls_H of device %d group %d must be a finite nonnegative scalar.', ...
            deviceIndex, groupIndex);
    end
    if isfield(g, 'Lser_ohm') && ...
            ~isempty(g.Lser_ohm) && ...
            ~is_nonnegative_finite_vector(g.Lser_ohm, 11)
        error('acload_relay:InvalidInductorResistance', ...
            ['Lser_ohm of device %d group %d must contain 11' ...
            ' finite nonnegative values.'], deviceIndex, groupIndex);
    end
    if (~isfield(g, 'Lser_ohm') || isempty(g.Lser_ohm)) && ...
            isfield(g, 'Rser_ohm') && ...
            ~is_positive_finite_scalar(g.Rser_ohm)
        error('acload_relay:InvalidSeriesResistance', ...
            'Rser_ohm of device %d group %d must be a finite positive scalar.', ...
            deviceIndex, groupIndex);
    end
end
end

function tf = is_positive_finite_scalar(x)
tf = isnumeric(x) && isreal(x) && isscalar(x) && ...
    ~isnan(x) && ~isinf(x) && x > 0;
end

function tf = is_nonnegative_finite_scalar(x)
tf = isnumeric(x) && isreal(x) && isscalar(x) && ...
    ~isnan(x) && ~isinf(x) && x >= 0;
end

function tf = is_positive_integer_scalar(x)
tf = is_positive_finite_scalar(x) && x == fix(x);
end

function tf = is_positive_finite_vector(x, expectedCount)
tf = isnumeric(x) && isreal(x) && ...
    isvector(x) && numel(x) == expectedCount && ...
    all(~isnan(x(:))) && all(~isinf(x(:))) && ...
    all(x(:) > 0);
end

function tf = is_nonnegative_finite_vector(x, expectedCount)
tf = isnumeric(x) && isreal(x) && ...
    isvector(x) && numel(x) == expectedCount && ...
    all(~isnan(x(:))) && all(~isinf(x(:))) && ...
    all(x(:) >= 0);
end

% function states = relay_state_names(closedMask)
% % 将逻辑继电器状态转换成 'CLOSED'/'OPEN' 字符单元数组。
% states = repmat({'OPEN'}, size(closedMask));
% states(closedMask) = ...
%     repmat({'CLOSED'}, 1, nnz(closedMask));
% end
%
% function name = get_device_name(device, fallbackIndex)
% if isfield(device, 'name') && ~isempty(device.name)
%     name = device.name;
% else
%     name = sprintf('Device %d', fallbackIndex);
% end
% end
function frame = acload_frame(data, packetCount)
%ACLOAD_FRAME 将16字节继电器控制数据域封装为完整的上位机控制帧
%
% 用法：
%   frame = acload_frame(data)
%   frame = acload_frame(data, packetCount)
%
% 输入：
%   data        16字节控制数据域（uint8或可转换为uint8的整数向量）
%               顺序为通信组1、组2、组3、组4，每组4字节，小端序。
%   packetCount 可选，包计数0~255；省略时默认为0。
%
% 输出：
%   frame       1×22 uint8完整控制帧：
%               AA 55 50 12 packetCount data(16B) checksum
%
% 校验和：
%   按协议，仅对帧头至包计数（前5字节）求算术和，取低8位。
%
% 注意：
%   data应由 acload_relay 的第二个输出参数生成，例如：
%       [results, data] = acload_relay(1);
%       frame = acload_frame(data(1,:), 0);

if nargin < 1
    error('acload_frame:MissingData', 'The 16-byte control data field data must be provided.');
end
if nargin < 2 || isempty(packetCount)
    packetCount = 0;
end
if ~isnumeric(data) || ~isreal(data) || ~isvector(data) || numel(data) ~= 16
    error('acload_frame:InvalidData', ...
        'data must be a real numeric vector with 16 elements.');
end
if any(~isfinite(double(data(:)))) || ...
        any(double(data(:)) < 0) || any(double(data(:)) > 255) || ...
        any(double(data(:)) ~= fix(double(data(:))))
    error('acload_frame:InvalidDataValue', ...
        'Each element of data must be an integer in the range 0-255.');
end
if ~isnumeric(packetCount) || ~isreal(packetCount) || ...
        ~isscalar(packetCount) || ~isfinite(double(packetCount)) || ...
        packetCount < 0 || packetCount > 255 || packetCount ~= fix(packetCount)
    error('acload_frame:InvalidPacketCount', ...
        'packetCount must be an integer in the range 0-255.');
end

data = uint8(reshape(data, 1, 16));
packetCount = uint8(packetCount);

% 固定帧头、帧ID、信息长度和包计数。
header = uint8([hex2dec('55'), hex2dec('AA'), ...
    hex2dec('50'), hex2dec('12'), packetCount]);

% 完整帧前21字节：头部5字节 + 数据域16字节。
frameWithoutChecksum = [header, data];

% 协议定义：校验从帧头至包计数，即只累加前5字节。
checksum = uint8(mod(sum(uint16(header)), 256));

% 总长度22字节。
frame = [frameWithoutChecksum, checksum];

% 打印完整帧数据。
% fprintf('\n--- 完整控制帧（%d字节）---\n', numel(frame));
% fprintf('  ');
% fprintf('%02X ', frame);
% fprintf('\n');
% fprintf('  帧头: %02X %02X  帧ID: %02X  长度: %02X  包计数: %02X\n', ...
%     frame(1), frame(2), frame(3), frame(4), frame(5));
% fprintf('  数据域: ');
% fprintf('%02X ', frame(6:21));
% fprintf('\n');
% fprintf('  校验和: %02X\n', frame(22));
end

== matlab function hk_ac_elec_load_rt_2024b/Subsystem/MATLAB Function ==
  data: clickStatus input; deviceId output
function deviceId = calc_deviceId(clickStatus)

% 由 clickStatus 的变化下标（从 1 开始）自动推断设备编号，无需外部输入 deviceId。
% clickStatus(k) 相对上一次发生变化，即表示第 k 台设备被点击；
% 一次只处理一个设备，多个元素同时变化时取下标最小的那个；
% 若本次没有检测到变化，沿用上一次的设备编号。
numDevices=2;
persistent prevStatus lastDeviceId
if isempty(prevStatus)
    prevStatus = zeros(1, numDevices);   % 与 Detect Change 的 vinit=[0,0] 一致
end
if isempty(lastDeviceId)
    lastDeviceId = 1;
end
deviceId = lastDeviceId;
found = false;
for k = 1:numDevices
    if clickStatus(k) ~= prevStatus(k) && ~found
        deviceId = k;
        found = true;
    end
end
lastDeviceId = deviceId;
for k = 1:numDevices
    prevStatus(k) = clickStatus(k);
end
